simulink model "XY_1_pen_sim"  (R2024b)
settings: Solver=ode4  StartTime=0.0  StopTime=T_run  FixedStep=Ts_plant  RelTol=1e-3
StopFcn:
  | XY_stop
values from neighbouring files (symbols this model uses):
  alpha_s = 0    [XY_setup.m]
  anim_Ts = 0.2    [XY_setup.m]
  animate = 1    [XY_1_pen_sim_run.m]    (also in XY_compare.m = 0; XY_run_all.m; XY_setup.m)
  B_eff = 0.30    (= 0.3)    [XY_setup.m]
  b_trk = 0.28    [XY_setup.m]
  d_reach = 0.03    [XY_setup.m]
  db_v = 47    [XY_setup.m]
  db_w = 20    [XY_setup.m]
  dist_p = [slip_k; wob_amp; wob_f]    [XY_setup.m]
  dyn_p = [m_r; l_trk; b_trk; mu_l; mu_t; N_mag; g_acc]    [XY_setup.m]
  F_max = 200    [XY_setup.m]
  imu_drift = deg2rad(0.02)    [XY_setup.m]
  imu_sigma = deg2rad(0.3)    [XY_setup.m]
  imu_Ts = 0.01    [XY_setup.m]
  K_c = 0    [XY_setup.m]
  K_ci = 0    [XY_setup.m]
  K_dist = 1.0    (= 1)    [XY_setup.m]
  K_ptheta = 1.4    [XY_setup.m]
  k_pwm = v_full/(400 - pwm_dz)    (= 0.000540540540541)    [XY_setup.m]
  K_px = 0.3    [XY_setup.m]
  K_py = 5.0    (= 5)    [XY_setup.m]
  K_yaw = 2.0    (= 2)    [XY_setup.m]
  Ki_v = 15000    [XY_setup.m]
  Ki_w = 15000    [XY_setup.m]
  Kp_v = 1500    [XY_setup.m]
  Kp_w = 1500    [XY_setup.m]
  L_r = sqrt((l_trk^2 + b_trk^2)/12)    [XY_setup.m]
  line_post = 0.04    [XY_setup.m]
  line_pre = 0.06    [XY_setup.m]
  pen_A = [-0.70; 0.30]    [XY_setup.m]
  pen_B = [ 0.50; 0.30]    [XY_setup.m]
  pen_d = r_pen0 - r_tag    [XY_setup.m]
  psi0 = pi/2    (= 1.57079632679)    [XY_setup.m]
  pwm_dz = 30    [XY_setup.m]
  q0 = [-0.85; 0.10; pi/2]    [XY_setup.m]
  q0c = [q0(1:2) - [cos(q0(3)) -sin(q0(3)); sin(q0(3)) cos(q0(3))] * r_tag; q0(3)]    [XY_setup.m]
  r_tag = [-0.080;  0.060]    [XY_setup.m]
  stage_acc = 500    [XY_setup.m]
  stage_c = stage_travel/2    (= 50.8)    [XY_setup.m]
  stage_cmd_Ts = 0.04    [XY_setup.m]
  stage_delay = 0.01    [XY_setup.m]
  stage_Fv_F = [32 32 29 26.5 25 22  20 17.5 14  9]    [XY_setup.m]
  stage_Fv_v = [0  2  7  13  20  32  45  60  80  104]    [XY_setup.m]
  stage_travel = 101.6    [XY_setup.m]
  stage_Ts = 0.05    [XY_setup.m]
  stage_vcmd = 0.8*stage_vmax    (= 83.2)    [XY_setup.m]
  stage_vmax = 104    [XY_setup.m]
  stg_p = [m_sx; m_sy; c_s; Kp_s; Kd_s; Ki_s; g_acc]    [XY_compare.m]    (also in XY_setup.m)
  tau_pred = 0    [XY_setup.m]
  th_tol = deg2rad(1)    [XY_setup.m]
  trk_A = -eye(2)/tau_trk    [XY_setup.m]
  trk_B = eye(2)/tau_trk    [XY_setup.m]
  trk_C = eye(2)    [XY_setup.m]
  trk_D = zeros(2)    [XY_setup.m]
  Ts_ctrl = 0.01    [XY_setup.m]
  v_full = 0.20    (= 0.2)    [XY_setup.m]
  v_max = 0.20    (= 0.2)    [XY_setup.m]
  v_ref = 0.03    [XY_setup.m]
  w_full = 2*k_pwm*(400 - db_w)/B_eff    (= 1.36936936937)    [XY_setup.m]
  w_max = deg2rad(45)    [XY_setup.m]
  x = c(1) + s(1)/2*[-1 1 1 -1 -1 1 1 -1]    [XY_animate.m]
  x_s0 = [stage_c; stage_c; 0; 0; 0; 0] .* [1e-3; 1e-3; 1; 1; 1; 1]    [XY_setup.m]
  x_t0 = [stage_c; stage_c; 0; 0]    [XY_setup.m]
  y = c(2) + s(2)/2*[-1 -1 1 1 -1 -1 1 1]    [XY_animate.m]    (also in build_xy_models.m = q(2))
  zk_delay = 0.05    [XY_setup.m]
  zk_sigma = 0.0010    (= 0.001)    [XY_setup.m]
  zk_Ts = 0.05    [XY_setup.m]
  zk_xsign = -1    [XY_setup.m]
  zk_ywall = 0.02    [XY_setup.m]
undefined symbols (not defined in the file or in its folder): orientation, point, quaternion, twist
libraries: ros2lib x20, simulink x4, slpidlib x2
(part 2 of 2)

== matlab function XY_1_pen_sim/PenCtrl/PenComp ==
  data: lineAB input; s_cmd output; mode input; pose input; pen_d input; stage_c input; pen_on output; sigma output
function [s_cmd, pen_on, sigma] = PenComp(lineAB, mode, pose, pen_d, stage_c)
% PenComp : 펜 기구학 보상. 펜이 직선 위에 오도록 스테이지 위치 명령을 계산한다
% PenComp : pen kinematic compensation. Computes the stage position command that puts the pen on the line
% 입력 / Inputs
%   lineAB  [4x1, m]   [A; B] 펜이 그릴 직선, 벽면 좌표 (x 오른쪽, y 위) / pen line in wall coordinates (x right, y up)
%   mode    [-]        미션 모드. 3 (직선 추종) 일 때만 보상 / mission mode; compensates only in mode 3
%   pose    [3x1: m, m, rad]  측정 태그 자세 [x; y; psi] (Nav) / measured tag pose
%   pen_d   [2x1, m]   태그 -> 펜 레버암, 바디 좌표 [x_B; y_B], 스테이지 중앙일 때 (= d)
%                      tag-to-pen lever arm in body axes, with the stage centred (= d)
%   stage_c [mm]       스테이지 중앙 (50.8, 두 축 같음) / stage centre (50.8 on both axes)
% 출력 / Outputs
%   s_cmd  [2x1, mm]   스테이지 목표 [X; Y] (X = x_B 전진 축, Y = y_B 왼쪽 축), 0-101.6
%                      stage target [X; Y] (X along x_B forward, Y along y_B left) -> /stage/target_pos
%   pen_on [0/1]       1 = 펜 다운 (펜 목표가 A 와 B 사이) / 1 = pen down (pen target between A and B)
%   sigma  [m]         직선 위 진행 거리 (A 에서 0, B 에서 L) / distance travelled along the line
% 원리 / Principle
%   펜 = 태그 + R(psi) (pen_d + (s - s_c)/1000) 을 s 에 대해 푼다. /1000 은 mm -> m.
%   Solve  pen = tag + R(psi) (pen_d + (s - s_c)/1000)  for s.  The 1000 converts m to mm.
%   p_des : 스테이지 중앙일 때 펜 위치 c0 를 직선에 내린 수선의 발
%           foot of the perpendicular from c0 (pen with the stage centred) to the line
%   진행 방향은 로봇이 맡고, 스테이지는 직선과의 어긋남(횡오차 + heading 오차)만 지운다
%   The robot provides the motion along the line; the stage removes only the offset from the line.
A = lineAB(1:2);  B = lineAB(3:4);
L = norm(B - A);  u = (B - A) / max(L, 1e-9);
pT = pose(1:2);
R  = [cos(pose(3)) -sin(pose(3)); sin(pose(3)) cos(pose(3))];
pc = pT + R * pen_d;                 % 스테이지 중앙일 때 펜 위치 / pen position with the stage centred
sigma = dot(u, pc - A);              % 직선 위 진행 거리 / distance along the line
pen_on = 0;
s_cmd = [stage_c; stage_c];
if round(mode) == 3
    % 직선 구간에 들어서면 펜을 내리기 전부터 스테이지를 미리 보낸다 (시작 과도 제거)
    % p_des 는 직선 위 수선의 발 (A, B 로 자르지 않는다): 진행 방향은 로봇이 맡고
    % 스테이지는 직선에서 벗어난 만큼만 지운다. A 로 자르면 펜이 A 앞에 있을 때
    % 남은 진행 거리(line_pre = 60 mm)까지 스테이지가 메우려 해서 행정 끝에 닿는다
%   On entering the line segment the stage is sent ahead even before pen down (removes the start transient).
%   p_des is the foot of the perpendicular on the line (not clipped to A, B): the robot provides the motion
%   along the line and the stage removes only the offset. Clipping to A would make the stage try to cover
%   the remaining run-in (line_pre = 60 mm) while the pen is before A, hitting the end of travel
    p_des = A + sigma * u;
    e_b = R' * (p_des - pT) - pen_d;   % 바디 좌표 펜 이동량 [m] / pen displacement in body frame [m]
    s_cmd = stage_c + 1000 * e_b;
    pen_on = double(sigma >= 0 && sigma <= L);
end

== matlab function XY_1_pen_sim/RobotPlant/EscInv ==
  data: motor_pwm input; v_trk_cmd output; pwm_dz input; k_pwm input
function v_trk_cmd = EscInv(motor_pwm, pwm_dz, k_pwm)
% EscInv : 가상 ESC. PWM -> 궤도 속도 명령 (calc_pwm 의 역) / virtual ESC: PWM -> track speed command
% 입력 / Inputs
%   motor_pwm [2x1, count] /motor_pwm [왼쪽; 오른쪽] / [left; right]
%   pwm_dz [count] ESC 데드존 (30) / ESC dead zone;   k_pwm [m/s per count] 기울기 / slope
% 출력 / Output
%   v_trk_cmd [2x1, m/s]  [vL; vR] 궤도 속도 명령 / track speed commands
% 원리: 우측 반전 해제 -> 데드존 -> count 를 속도로 / undo the right-motor inversion, dead zone, scale
pL =  (motor_pwm(1) - 1500);
pR = -(motor_pwm(2) - 1500);
v_trk_cmd = k_pwm * [sign(pL) * max(0, abs(pL) - pwm_dz);
                     sign(pR) * max(0, abs(pR) - pwm_dz)];

== matlab function XY_1_pen_sim/RobotPlant/SpeedErr ==
  data: v_trk input; e_v output; V_act input; B_eff input; L_r input; e_Lw output
function [e_v, e_Lw] = SpeedErr(v_trk, V_act, B_eff, L_r)
% SpeedErr (운동모델) : 궤도 속도 명령 -> 차체 속도 오차. 6WP 와 같이 둘째 성분은 L*omega 단위
% SpeedErr (plant)    : track speed command -> body speed error; 2nd component in L*omega units as in 6WP
% 입력 / Inputs
%   v_trk [2x1, m/s]  지연을 거친 궤도 속도 명령 [vL; vR] / lagged track speed commands
%   V_act [2x1: m/s, rad/s]  실제 차체 속도 [v; omega] / actual body speed
%   B_eff [m]  조향 유효 궤도 간격 / effective track spacing;   L_r [m]  관성 반경 / radius of gyration
% 출력 / Outputs
%   e_v [m/s] = (vL+vR)/2 - v,   e_Lw [m/s] = L_r ((vR-vL)/B_eff - omega)
v_c = 0.5 * (v_trk(1) + v_trk(2));
w_c = (v_trk(2) - v_trk(1)) / B_eff;
e_v  = v_c - V_act(1);
e_Lw = L_r * (w_c - V_act(2));

== matlab function XY_1_pen_sim/RobotPlant/Control_allocation ==
  data: tau_X input; Fr output; tau_N input; b_trk input; L_r input; Fl output
function [Fr, Fl] = Control_allocation(tau_X, tau_N, b_trk, L_r)
% Control_allocation : 차체 힘·모멘트 -> 좌우 궤도 구동력 (6WP_sim 과 같은 식)
% Control_allocation : body force and moment -> right/left track forces (as in 6WP_sim)
% 입력 / Inputs : tau_X [N] 전진 힘 / surge force;  tau_N [N] 요 모멘트/L / yaw moment divided by L
%                 b_trk [m] 궤도 간격 / track spacing;  L_r [m]
% 출력 / Outputs: Fr, Fl [N] 오른쪽·왼쪽 궤도 구동력 / right and left track forces
% 원리: [tau_X; tau_N] = [1 1; b/2L -b/2L] [Fr; Fl] 를 푼다 / solve this 2x2 system
B_tilde = [1, 1; b_trk/(2*L_r), -b_trk/(2*L_r)];
F = B_tilde \ [tau_X; tau_N];
Fr = F(1);  Fl = F(2);

== matlab function XY_1_pen_sim/RobotPlant/compute_u ==
  data: V_act input; u output; alpha_s input
function u = compute_u(V_act, alpha_s)
% compute_u (6WP_sim) : 회전 중심(ICR)의 길이방향 이동량 / longitudinal shift of the ICR
% 입력 / Inputs : V_act [m/s, rad/s];  alpha_s [rad] ICR 이동각 (0 이면 u = 0) / ICR shift angle
% 출력 / Output : u [m]
R_turn = abs(V_act(1) / max(0.01, abs(V_act(2))));
u = -sign(V_act(2)) * R_turn * sin(alpha_s);

== matlab function XY_1_pen_sim/RobotPlant/Dynamics ==
  data: q input; V_act input; u input; V_dot output; u_dot input; Fr input; Fl input; dyn_p input
function V_dot = Dynamics(q, V_act, u, u_dot, Fr, Fl, dyn_p)
% Dynamics : 궤도차량 동역학 (Zou 2018), 벽면판 / tracked-vehicle dynamics (Zou 2018), wall version
% 입력 / Inputs
%   q [3x1: m, m, rad]  로봇 중심 자세 / robot centre pose;  V_act [2x1: m/s, rad/s] [v; omega]
%   u [m], u_dot [m/s]  ICR 이동량과 그 미분 / ICR shift and its rate
%   Fr, Fl [N]  궤도 구동력 / track forces
%   dyn_p = [m kg; l m; b m; mu_l -; mu_t -; N_mag N; g m/s^2]
% 출력 / Output : V_dot [2x1: m/s^2, rad/s^2]
% 원리 / Principle : M~ nu_dot + C~ nu + S^T (f1 + f2) = B~ tau + S^T f_g,  nu = [v; L omega]
% 6WP_sim Dynamics 와 같은 식 (궤도차량 동역학, 논문 Table 1 모델). 벽면판에서 바꾼 점:
%  (1) 바닥 하중 W -> 자석 흡착력 N_mag : 벽에서 마찰을 만드는 수직력
%  (2) 중력 f_g = [0; -m g; 0] 추가    : 벽면 y = 위
%  (3) 회전 저항 Mr 는 회전을 막는 쪽으로 (l^2/4 - u^2). 6WP 식 (u^2 - l^2/4) 은
%      u = 0 근처에서 회전을 돕는 부호가 되어 헤딩 떨림(stick-slip)을 만든다
%  (4) sign() -> tanh(./eps) : 정지 근처 수치 떨림 방지
% Same equations as 6WP_sim Dynamics (tracked-vehicle dynamics, Table 1 model of the paper). Wall-version changes:
%  (1) ground load W -> magnetic adhesion N_mag : the normal force that creates friction on the wall
%  (2) gravity f_g = [0; -m g; 0] added  : wall y = up
%  (3) turning resistance Mr opposes rotation, (l^2/4 - u^2). The 6WP form (u^2 - l^2/4) assists
%      rotation near u = 0 and causes heading stick-slip
%  (4) sign() -> tanh(./eps) : avoids numerical chatter near standstill
m = dyn_p(1); l = dyn_p(2); b = dyn_p(3); mu_l = dyn_p(4); mu_t = dyn_p(5); N = dyn_p(6); g = dyn_p(7);
L = sqrt((l^2 + b^2)/12);
B_tilde = [1, 1; b/(2*L), -b/(2*L)];
B_tau = B_tilde * [Fr; Fl];
theta = q(3);  v = V_act(1);  omega = V_act(2);
M_mat = m * eye(3);
Rl = mu_l * N / 2;
f1_vec = [2*Rl*cos(theta); 2*Rl*sin(theta); 0] * tanh(v/0.005);
Fy = 2 * tanh(omega/0.01) * mu_t * u * (N / l);
Mr = tanh(omega/0.01) * mu_t * (N / l) * (l^2/4 - u^2);
f2_vec = [Fy*sin(theta); -Fy*cos(theta); Mr/L];
f_g = [0; -m*g; 0];
S_mat = [cos(theta), (u/L)*sin(theta); sin(theta), -(u/L)*cos(theta); 0, 1];
S_dot = [-omega*sin(theta), (u_dot/L)*sin(theta) + (u*omega/L)*cos(theta);
          omega*cos(theta), -(u_dot/L)*cos(theta) + (u*omega/L)*sin(theta); 0, 0];
M_tilde = S_mat' * M_mat * S_mat;
C_tilde = S_mat' * M_mat * S_dot;
V_dot = M_tilde \ (B_tau - C_tilde*[v; L*omega] - S_mat'*f1_vec - S_mat'*f2_vec + S_mat'*f_g);
V_dot(2) = V_dot(2) / L;          % [v_dot; omega_dot]

== matlab function XY_1_pen_sim/Mission/Guards ==
  data: pose input; dist_start output; pen_A input; pen_B input; pen_d input; line_pre input; line_post input; r_tag input; th_err output; along_rem output
function [dist_start, th_err, along_rem] = Guards(pose, pen_A, pen_B, pen_d, line_pre, line_post, r_tag)
% Guards : Stateflow 전이 조건에 쓸 거리·각 (실기 Chart 의 dist, th_err, dist_to_WP2 와 같은 뜻)
% Guards : distances and angle used by the Stateflow transitions (dist, th_err, dist_to_WP2 of the real Chart)
% 입력 / Inputs
%   pose         [3x1: m, m, rad] 측정 태그 자세 [x; y; psi] / measured tag pose
%   pen_A, pen_B [2x1, m]   펜이 그릴 직선의 시작·끝 (벽면) / start and end of the pen line (wall)
%   pen_d        [2x1, m]   태그 -> 펜 레버암, 바디 좌표, 스테이지 중앙일 때 / tag-to-pen lever arm, body frame, stage centred
%   line_pre, line_post [m] 직선 앞뒤로 로봇이 더 가는 거리 / run-in and run-out lengths of the robot segment
%   r_tag        [2x1, m]   로봇 중심 -> 태그, 바디 좌표 / robot centre to tag, body frame
% 출력 / Outputs
%   dist_start [m]   추정 중심과 출발 중심 cA 의 거리 (모드 1 -> 2) / estimated centre to start centre cA (mode 1 -> 2)
%   th_err     [rad] 직선 방향 - heading, [-pi, pi] (모드 2 -> 3) / line direction minus heading (mode 2 -> 3)
%   along_rem  [m]   태그에서 로봇 끝점 rB 까지 남은 진행 거리 (모드 3 -> 4) / distance left to rB along the line (mode 3 -> 4)
th = atan2(pen_B(2) - pen_A(2), pen_B(1) - pen_A(1));   % 펜 직선 방향 / pen line direction
u  = [cos(th); sin(th)];
R  = [cos(th) -sin(th); sin(th) cos(th)];
% 로봇(태그)이 따라갈 선 = 펜 직선을 R*pen_d 만큼 옮긴 것 (스테이지 중앙일 때 펜이 직선 위)
% Line the robot (tag) follows = pen line shifted by R*pen_d (pen on the line when the stage is centred)
rA = pen_A - R*pen_d - u*line_pre;    % 로봇 출발점 (펜이 A 에 닿기 line_pre 전) / robot start (line_pre before the pen reaches A)
rB = pen_B - R*pen_d + u*line_post;   % 로봇 끝점 / robot end point
% 제자리 회전은 중심 둘레로 돈다: 회전 뒤 태그가 rA 에 오려면 중심이 cA 에 있어야 한다
% In-place turns pivot about the centre: for the tag to end at rA the centre must be at cA
cA = rA - R*r_tag;
p = pose(1:2);
Rp = [cos(pose(3)) -sin(pose(3)); sin(pose(3)) cos(pose(3))];
dist_start = norm(cA - (p - Rp*r_tag));                        % 중심과 출발 중심 cA 의 거리 / centre to start centre cA
th_err     = atan2(sin(th - pose(3)), cos(th - pose(3)));      % 직선 방향 오차 / line direction error
along_rem  = dot(rB - p, u);                                   % 끝점까지 남은 진행 거리 / distance left to the end point

== matlab function XY_1_pen_sim/RobotPlant/Kinematics ==
  data: V_act input; q input; u input; q_dot output; t input; dist_p input
function q_dot = Kinematics(V_act, q, u, t, dist_p)
% Kinematics : 차체 속도 -> 중심 자세 변화율 (+ 벽면 외란) / body speed -> centre pose rate (+ wall disturbance)
% 입력 / Inputs : V_act [m/s, rad/s];  q [m, m, rad] 중심 자세 / centre pose;  u [m];  t [s]
%                 dist_p = [slip_k -; 요철 진폭 A rad / wobble amplitude; 주파수 f Hz / frequency]
% 출력 / Output : q_dot [3x1: m/s, m/s, rad/s]
% 6WP_sim Kinematics: q_dot = S_mat * [v; L*omega]  (여기서는 q(3) = psi 로 정리)
% 벽면 외란 (실기 영상·ZeroKey 로그에서 본 현상, [실측 필요]):
%   자석 궤도 크리프 : 이동 속도의 slip_k 배만큼 중력 방향(-y) 으로 밀린다
%   궤도 요철        : heading 이 두 주파수로 조금씩 흔들린다
% 6WP_sim Kinematics: q_dot = S_mat * [v; L*omega]  (written here with q(3) = psi)
% Wall disturbances (seen in real robot videos and ZeroKey logs, [measurement needed]):
%   magnetic track creep : pushed toward gravity (-y) by slip_k times the travel speed
%   track unevenness     : heading wobbles slightly at two frequencies
theta = q(3);  v = V_act(1);  omega = V_act(2);
slip_k = dist_p(1);  A = dist_p(2);  f = dist_p(3);
wob = A*2*pi*f*cos(2*pi*f*t) + 0.5*A*2*pi*(2.3*f)*cos(2*pi*(2.3*f)*t + 1.0);
q_dot = [v*cos(theta) + u*omega*sin(theta);
         v*sin(theta) - u*omega*cos(theta) - slip_k*abs(v);
         omega + wob];

== matlab function XY_1_pen_sim/RobotPlant/TagPoint ==
  data: q_c input; q_tag output; r_tag input
function q_tag = TagPoint(q_c, r_tag)
% TagPoint : 입력 q_c [m, m, rad] 중심 자세, r_tag [2x1, m] -> 출력 q_tag [m, m, rad] 태그 자세 (= q_true)
% TagPoint : input centre pose q_c and r_tag -> output tag pose q_tag (= q_true)
% 중심 -> 태그: p = c + R(psi) r_tag. 회전하면 태그는 반경 |r_tag| 원호를 그린다
% Centre -> tag: p = c + R(psi) r_tag. While turning the tag moves on an arc of radius |r_tag|
R = [cos(q_c(3)) -sin(q_c(3)); sin(q_c(3)) cos(q_c(3))];
q_tag = [q_c(1:2) + R * r_tag; q_c(3)];

== matlab function XY_1_pen_sim/Sensors/ZkWorld ==
  data: q_true input; zk output; zk_ywall input; noise input; zk_xsign input
function zk = ZkWorld(q_true, zk_ywall, noise, zk_xsign)
% ZkWorld : 가상 ZeroKey 위치 / virtual ZeroKey position
% 입력 / Inputs : q_true [m, m, rad] 참 태그 자세 / true tag pose;  zk_ywall [m] 벽 법선 오프셋 / wall-normal offset
%                 noise [3x1, m] 백색 잡음 (sigma 1 mm) / white noise
% 출력 / Output : zk [3x1, m] 월드 [x; y; z] -> 지연 50 ms -> 20 Hz -> /zerokey/position
% 벽면 (x, y) -> ZeroKey 월드 좌표 (x = zk_xsign * 벽면 x, y = 벽 법선 오프셋, z = 벽면 y) + 측정 잡음
% Wall (x, y) -> ZeroKey world (x = zk_xsign * wall x, y = wall-normal offset, z = wall y) + noise
zk = [zk_xsign * q_true(1); zk_ywall; q_true(2)] + noise(:);

== matlab function XY_1_pen_sim/Sensors/ZkVel ==
  data: q_true input; zkv output; V_true input; r_tag input; zk_xsign input
function zkv = ZkVel(q_true, V_true, r_tag, zk_xsign)
% ZkVel : 입력 q_true [m, m, rad], V_true [m/s, rad/s], r_tag [m] -> 출력 zkv [3x1, m/s] -> /zerokey/vel
% ZkVel : inputs q_true, V_true, r_tag -> output zkv [3x1, m/s] world velocity -> /zerokey/vel
% ZeroKey 속도 (월드): x = zk_xsign * 벽면 x, z = 벽면 y. 태그 속도 = 중심 속도 + omega J R r_tag
% ZeroKey velocity (world): x = zk_xsign * wall x, z = wall y. Tag velocity = centre velocity + omega J R r_tag
psi = q_true(3);  R = [cos(psi) -sin(psi); sin(psi) cos(psi)];
pd = V_true(1) * [cos(psi); sin(psi)] + V_true(2) * [0 -1; 1 0] * R * r_tag;
zkv = [zk_xsign * pd(1); 0; pd(2)];

== matlab function XY_1_pen_sim/Sensors/ImuQuat ==
  data: q_true input; quat output; t input; imu_drift input; noise input
function quat = ImuQuat(q_true, t, imu_drift, noise)
% ImuQuat : 입력 q_true [m, m, rad], t [s], imu_drift [rad/s], noise [rad] -> 출력 quat [4x1] (w,x,y,z) -> /imu/data
% ImuQuat : inputs true pose, time, drift rate, noise -> output attitude quaternion -> /imu/data
% IMU 요각 = 참 heading + 드리프트 + 잡음 -> 쿼터니언 (6WP_sim Euler2Quat 와 같은 식)
% IMU yaw = true heading + drift + noise -> quaternion (same as 6WP_sim Euler2Quat)
psi = q_true(3) + imu_drift * t + noise;
quat = [cos(psi/2); 0; 0; sin(psi/2)];

== matlab function XY_1_pen_sim/Sensors/ZkQuat ==
  data: q_true input; quat output; noise input
function quat = ZkQuat(q_true, noise)
% ZkQuat : 입력 q_true, noise [rad] -> 출력 quat [4x1] -> /zerokey/orientation (이 제어기는 쓰지 않음)
% ZkQuat : output quaternion -> /zerokey/orientation (not used by this controller, kept for the real models)
% ZeroKey INS 요각 = 참 heading + 잡음 (드리프트 없음, 대신 IMU 보다 잡음이 크다) -> 쿼터니언
% ZeroKey INS yaw = true heading + noise (no drift, but noisier than the IMU) -> quaternion
psi = q_true(3) + noise;
quat = [cos(psi/2); 0; 0; sin(psi/2)];

== matlab function XY_1_pen_sim/StagePlant/ZaberTraj ==
  data: s_goal input; x_t_dot output; x_t input; stage_vmax input; stage_acc input; stage_travel input
function x_t_dot = ZaberTraj(s_goal, x_t, stage_vmax, stage_acc, stage_travel)
% ZaberTraj : Zaber 펌웨어 궤적 생성기의 모델 (사용자가 바꿀 수 없는 상용 부분)
% ZaberTraj : model of the Zaber firmware trajectory generator (commercial, not ours to change)
% 입력 / Inputs : s_goal [2x1, mm] move abs 목표 / move abs target;  x_t [4x1: mm, mm, mm/s, mm/s]
%                 stage_vmax [mm/s] maxspeed;  stage_acc [mm/s^2] accel;  stage_travel [mm] 행정 / travel
% 출력 / Output : x_t_dot [4x1: mm/s, mm/s, mm/s^2, mm/s^2]
% Zaber 펌웨어의 move abs 궤적 (두 축 따로).  상태 x_t = [s_t(2) mm; v_t(2) mm/s]
%   목표까지 남은 거리에서 멈출 수 있는 속도 sqrt(2 a |e|) 와 maxspeed 중 작은 값으로 간다
%   (가속·감속 한계 = accel 설정).  새 move abs 가 오면 그 자리에서 목표만 바뀐다
% Zaber firmware move abs trajectory (each axis separately).  State x_t = [s_t(2) mm; v_t(2) mm/s]
%   Moves at the smaller of maxspeed and the speed sqrt(2 a |e|) that can still stop at the target
%   (acceleration/deceleration limit = accel setting).  A new move abs only changes the target in place
goal = min(max(s_goal(:), 0), stage_travel);
s = x_t(1:2);  v = x_t(3:4);
e = goal - s;
v_des = sign(e) .* min(stage_vmax, sqrt(2*stage_acc*abs(e)));
a = min(max(50*(v_des - v), -stage_acc), stage_acc);
x_t_dot = [v; a];

== matlab function XY_1_pen_sim/StagePlant/ZaberServo ==
  data: x_t input; x_dot output; x_s input; q_true input; stg_p input; Fv_v input; Fv_F input
function x_dot = ZaberServo(x_t, x_s, q_true, stg_p, Fv_v, Fv_F)
% ZaberServo : Zaber 내부 위치 서보 + 캐리지 질량의 모델 (상용 펌웨어, 명령만 줄 수 있음)
% ZaberServo : model of the internal Zaber position servo and carriage mass (commercial; command only)
% 입력 / Inputs : x_t [mm, mm/s] 궤적 / trajectory;  x_s [6x1: m, m, m/s, m/s, m s, m s] 캐리지 상태 / carriage state
%                 q_true [m, m, rad] (중력 방향 계산 / for the gravity direction)
%                 stg_p = [m_X kg; m_Y kg; c N s/m; Kp N/m (2); Kd N s/m (2); Ki N/(m s) (2); g m/s^2]
%                 Fv_v [mm/s], Fv_F [N]  추력-속도 곡선 / thrust-speed curve
% 출력 / Output : x_dot [6x1: m/s, m/s, m/s^2, m/s^2, m, m]
% Zaber X-LSM100B 두 축 (X = 아래 축, Y = 위 축).  상태 x_s = [s(2) m; v(2) m/s; 적분(2)]
%   스테퍼는 궤적을 단단한 스프링처럼 따라간다 -> 높은 대역의 위치 루프로 나타낸다
%   낼 수 있는 힘은 속도에 따라 줄어든다 (데이터시트 Thrust-Speed, B 형 24 V 곡선 Fv_v -> Fv_F)
%   X 축은 Y 축 스테이지 전체 + 펜 홀더를 민다 (m_sx > m_sy)
%   벽면 중력 [0; -g] 를 바디 좌표로 돌려 각 축에 m g 성분을 건다
% Two-axis Zaber X-LSM100B (X = lower axis, Y = upper axis).  State x_s = [s(2) m; v(2) m/s; integral(2)]
%   The stepper follows the trajectory like a stiff spring -> modelled as a high-bandwidth position loop
%   Available force drops with speed (datasheet Thrust-Speed, type B 24 V curve Fv_v -> Fv_F)
%   The X axis pushes the whole Y-axis stage + pen holder (m_sx > m_sy)
%   Wall gravity [0; -g] is rotated into the body frame and its m g component applied on each axis
m  = stg_p(1:2);  c = stg_p(3);
Kp = stg_p(4:5);  Kd = stg_p(6:7);  Ki = stg_p(8:9);  g = stg_p(10);
s = x_s(1:2);  v = x_s(3:4);  ie = x_s(5:6);
s_t = x_t(1:2)/1000;  v_t = x_t(3:4)/1000;
e = s_t - s;
F_av = interp1(Fv_v, Fv_F, min(abs(v)*1000, Fv_v(end)));   % 지금 속도에서 낼 수 있는 추력 [N] / thrust available at the current speed [N]
F = min(max(Kp.*e + Ki.*ie + Kd.*(v_t - v), -F_av), F_av);
psi = q_true(3);
g_b = [cos(psi) sin(psi); -sin(psi) cos(psi)] * [0; -g];
a = (F + m.*g_b - c*v) ./ m;
x_dot = [v; a; e];

== matlab function XY_1_pen_sim/StagePlant/Encoder ==
  data: x_s input; stage_pos output; stage_travel input
function stage_pos = Encoder(x_s, stage_travel)
% Encoder : 입력 x_s [m, m/s, m s], stage_travel [mm] -> 출력 stage_pos [2x1, mm] -> /stage/pos (20 Hz)
% Encoder : output = position reported by get pos [mm], clipped at the travel ends
% 내장 엔코더 위치 [mm] (get pos 가 돌려주는 값), 행정 끝에서 막힌다
stage_pos = min(max(1000 * x_s(1:2), 0), stage_travel);

== matlab function XY_1_pen_sim/PenTrace/PenTraceFcn ==
  data: q_true input; pen_true output; stage_pos input; lineAB input; pen_d input; stage_c input; pen_nocomp output; e_pen output; e_nocomp output
function [pen_true, pen_nocomp, e_pen, e_nocomp] = PenTraceFcn(q_true, stage_pos, lineAB, pen_d, stage_c)
% PenTraceFcn : 참값으로 계산한 펜 위치와 횡오차 (평가 전용, 제어기는 모름)
% PenTraceFcn : true pen position and cross error from true values (evaluation only)
% 입력 / Inputs : q_true [m, m, rad] 참 태그 자세 / true tag pose;  stage_pos [2x1, mm] 엔코더 / encoder;  lineAB [4x1, m];
%                 pen_d [2x1, m];  stage_c [mm]
% 출력 / Outputs: pen_true, pen_nocomp [2x1, m];  e_pen, e_nocomp [m]
% pen_true   : 스테이지가 실제로 움직인 결과의 펜 위치 [x; y] (벽면)
%              pen position [x; y] resulting from the actual stage motion (wall frame)
% pen_nocomp : 스테이지를 중앙에 고정했을 때 펜 위치 (보상 없음 비교)
%              pen position with the stage held at centre (no-compensation comparison)
% e_*        : 직선에 대한 부호 있는 횡오차 [m] (직선 진행방향의 왼쪽 +)
%              signed cross error to the line [m] (left of the line direction +)
A = lineAB(1:2);  B = lineAB(3:4);
u = (B - A) / max(norm(B - A), 1e-9);  n = [-u(2); u(1)];
pT = q_true(1:2);
R  = [cos(q_true(3)) -sin(q_true(3)); sin(q_true(3)) cos(q_true(3))];
pen_true   = pT + R * (pen_d + (stage_pos - stage_c) / 1000);
pen_nocomp = pT + R * pen_d;
e_pen    = dot(n, pen_true - A);
e_nocomp = dot(n, pen_nocomp - A);

== matlab function XY_1_pen_sim/Animate/AnimateFcn ==
  data: q_true input; ok output; pen_true input; pen_on input; stage_pos input; lineAB input; e_pen input; v_cmd input; w_cmd input; V_true input; mode input; t input; en input
function ok = AnimateFcn(q_true, pen_true, pen_on, stage_pos, lineAB, e_pen, v_cmd, w_cmd, V_true, mode, t, en)
%#codegen
% Live plot while the model runs. A MATLAB Function block cannot
% plot, so the drawing function is declared extrinsic: Simulink
% calls plain MATLAB instead of generating code for it.
coder.extrinsic('XY_animate');
ok = 1;
if en > 0.5
    XY_animate(q_true, pen_true, pen_on, stage_pos, lineAB, e_pen, v_cmd, w_cmd, V_true, mode, t);
end

== matlab function XY_1_pen_sim/Nav/NavFcn ==
  settings: updateMethod=DISCRETE  sampleTime=Ts_ctrl
  data: zerokey_position input; pose output; zerokey_vel input; imu_quat input; psi0 input; tau_pred input; zk_xsign input
function pose = NavFcn(zerokey_position, zerokey_vel, imu_quat, psi0, tau_pred, zk_xsign)
% NavFcn : 센서 토픽 -> 측정 자세 (항법)
% NavFcn : sensor topics -> measured pose (navigation)
% 입력 / Inputs
%   zerokey_position [3x1, m]   /zerokey/position point.(x,y,z). 태그 월드 좌표: x 벽 수평, y 벽 법선, z 높이
%                               tag world position: x horizontal, y wall normal, z height
%   zerokey_vel      [3x1, m/s] /zerokey/vel twist.linear.(x,y,z). 태그 월드 속도 / tag world velocity
%   imu_quat         [4x1, -]   /imu/data orientation (w,x,y,z). Xsens 자세 쿼터니언 / Xsens attitude quaternion
%   psi0             [1, rad]   출발 heading (오른쪽 0, 천장 pi/2) / initial heading (0 = right, pi/2 = up)
%   tau_pred         [1, s]     ZeroKey 지연 보상 시간 (0 = 끔) / ZeroKey latency compensation (0 = off)
%   zk_xsign         [-1 / +1]  ZeroKey x 방향: -1 = 벽 정면에서 왼쪽 +, +1 = 오른쪽 + / ZeroKey x: -1 left +, +1 right +
% 출력 / Output
%   pose [3x1: m, m, rad]  [x; y; psi] = 태그 벽면 위치 (x 오른쪽 +, y 위 +) + heading (x 축에서 반시계)
%                          [x; y; psi] = tag position on the wall (x right, y up) + heading (CCW from x)
% 원리 / Principle
%   벽면 x = zk_xsign * ZeroKey x, 벽면 y = ZeroKey z (REP-103 형: z 가 벽 바깥인 오른손 좌표계).
%   철판 벽에서는 자력계를 못 쓰므로 heading 은 첫 유효 샘플의 요각을 0 으로 잡은 상대 요각에 psi0 를 더한 값이다.
%   Wall x = zk_xsign * ZeroKey x, wall y = ZeroKey z (REP-103 style, right-handed with z out of the wall).
%   The steel wall disturbs the magnetometer, so heading is the yaw relative to the first valid sample, plus psi0.
persistent yaw0 ok
if isempty(ok), ok = false; yaw0 = 0; end
qw = imu_quat(1); qx = imu_quat(2); qy = imu_quat(3); qz = imu_quat(4);
yaw = atan2(2*(qw*qz + qx*qy), 1 - 2*(qy*qy + qz*qz));
if ~ok && (abs(qw) + abs(qx) + abs(qy) + abs(qz)) > 0.5
    yaw0 = yaw;  ok = true;
end
a = yaw - yaw0 + psi0;
pose = [zk_xsign * zerokey_position(1); zerokey_position(3); atan2(sin(a), cos(a))];
% ZeroKey 지연 보상 (tau_pred = 0 이면 끔): 측정 속도로 tau_pred 만큼 앞으로 내다본다
% ZeroKey latency compensation (off when tau_pred = 0): predicts ahead by tau_pred with the measured velocity
pose(1:2) = pose(1:2) + tau_pred * [zk_xsign * zerokey_vel(1); zerokey_vel(3)];

== stateflow chart XY_1_pen_sim/Mission/ModeChart ==
  settings: updateMethod=DISCRETE  sampleTime=Ts_ctrl
  state Goto_Start
    entry:
    mode = 1;
  state Turning
    entry:
    mode = 2;
  state Line_Tracking
    entry:
    mode = 3;
    t_line = t;
  state Stop_Destination
    entry:
    mode = 4;
  state Done
    entry:
    done = 1;
  (default) -> Goto_Start
  Goto_Start -> Turning : [dist_start < d_reach]
  Turning -> Line_Tracking : after(1.0,sec)[abs(th_err) < th_tol]
  Line_Tracking -> Stop_Destination : [along_rem < d_reach]
  Stop_Destination -> Done : after(2.0,sec)
  data: dist_start input; th_err input; along_rem input; t input; mode output double =1; t_line output double =0; done output double =0; d_reach parameter; th_tol parameter

== matlab function XY_1_pen_sim/Mission/Waypoints ==
  data: mode input; WP_prev output; pen_A input; pen_B input; pen_d input; line_pre input; line_post input; r_tag input; WP_target output; lineAB output
function [WP_prev, WP_target, lineAB] = Waypoints(mode, pen_A, pen_B, pen_d, line_pre, line_post, r_tag)
% Waypoints : 모드에 따라 로봇이 따라갈 선분을 낸다 (6WP waypoint_manager 역할)
% Waypoints : gives the segment the robot follows in each mode (role of the 6WP waypoint_manager)
% 입력 / Inputs
%   mode [-]  1 출발점 이동, 2 회전, 3 직선 추종, 4 정지, 5 종료 / 1 go to start, 2 turn, 3 line, 4 stop, 5 done
%   pen_A, pen_B, pen_d, line_pre, line_post, r_tag : Guards 와 같음 / same as Guards
% 출력 / Outputs
%   WP_prev   [2x1, m] 태그 선분 시작 rA (펜이 A 에 닿기 line_pre 전) / tag segment start rA
%   WP_target [2x1, m] 모드 1: 출발 중심 cA (중심 기준), 그 뒤: 태그 선분 끝 rB
%                      mode 1: start centre cA (centre-referenced); afterwards: tag segment end rB
%   lineAB    [4x1, m] [A; B] 펜 직선 (PenComp 로 간다) / pen line, sent to PenComp
% 원리 / Principle
%   스테이지가 중앙일 때 펜이 직선 위에 오도록, 태그가 갈 선분은 펜 직선을 R(theta_l) pen_d 만큼 옮긴 것이다.
%   The tag segment is the pen line shifted by -R(theta_l) pen_d, so that the pen is on the line when the stage is centred.
th = atan2(pen_B(2) - pen_A(2), pen_B(1) - pen_A(1));   % 펜 직선 방향 / pen line direction
u  = [cos(th); sin(th)];
R  = [cos(th) -sin(th); sin(th) cos(th)];
% 로봇(태그)이 따라갈 선 = 펜 직선을 R*pen_d 만큼 옮긴 것 (스테이지 중앙일 때 펜이 직선 위)
% Line the robot (tag) follows = pen line shifted by R*pen_d (pen on the line when the stage is centred)
rA = pen_A - R*pen_d - u*line_pre;    % 로봇 출발점 (펜이 A 에 닿기 line_pre 전) / robot start (line_pre before the pen reaches A)
rB = pen_B - R*pen_d + u*line_post;   % 로봇 끝점 / robot end point
% 제자리 회전은 중심 둘레로 돈다: 회전 뒤 태그가 rA 에 오려면 중심이 cA 에 있어야 한다
% In-place turns pivot about the centre: for the tag to end at rA the centre must be at cA
cA = rA - R*r_tag;
WP_prev = rA;
if round(mode) <= 1
    WP_target = cA;
else
    WP_target = rB;
end
lineAB = [pen_A; pen_B];

== matlab function XY_1_pen_sim/RobotCtrl/M1_GotoStart/Fcn1_GotoStart ==
  data: WP_target input; v output; pose input; K_dist input; K_yaw input; r_tag input; w output
function [v, w] = Goto_Start_Position(WP_target, pose, K_dist, K_yaw, r_tag)
% 모드 1 : 6WP_sim Goto_Start_Position, Method 2 (리아프노프형). 6WP 와 같이 로봇 중심을 목표로 보낸다
% Mode 1 : 6WP_sim Goto_Start_Position, Method 2. Drives the robot centre (as in 6WP_sim) to the target
% 입력 / Inputs
%   WP_target [2x1, m]   출발 중심 cA (벽면) / start centre cA (wall)
%   pose      [3x1: m, m, rad] 측정 태그 자세 / measured tag pose
%   K_dist    [1/s]  거리 게인 / distance gain;   K_yaw [1/s]  방향 게인 / bearing gain
%   r_tag     [2x1, m]  중심 -> 태그 (바디) / centre to tag (body)
% 출력 / Outputs
%   v [m/s]   전진 속도 명령 / forward speed command;   w [rad/s] 요 각속도 명령 (반시계 +) / yaw-rate command (CCW +)
% 원리 / Principle
%   v = K_dist rho max(0, cos a), w = K_yaw a + 0.5 sin a cos a. a = 목표 방위 - heading.
%   방향이 90 도 넘게 틀리면 서서 돌기만 한다 / turns on the spot while the bearing error exceeds 90 deg
c = pose(1:2) - [cos(pose(3)) -sin(pose(3)); sin(pose(3)) cos(pose(3))] * r_tag;   % 중심 추정 / centre estimate
err_x = WP_target(1) - c(1);  err_y = WP_target(2) - c(2);
dist = hypot(err_x, err_y);
target_th = atan2(err_y, err_x);
a = atan2(sin(target_th - pose(3)), cos(target_th - pose(3)));
v = K_dist * dist * max(0, cos(a));            % 방향이 맞을 때만 전진 / forward only when roughly aligned
w = K_yaw * a + 0.5 * sin(a) * cos(a);         % 비선형 감쇠항 / nonlinear damping term

== matlab function XY_1_pen_sim/RobotCtrl/M2_Turn/Fcn2_Turn ==
  data: WP_prev input; v output; WP_target input; pose input; K_yaw input; w output
function [v, w] = Turning_Straight_Mode(WP_prev, WP_target, pose, K_yaw)
% 모드 2 : 6WP_sim Turning_Straight_Mode — 제자리 회전으로 heading 을 직선 방향에 맞춘다
% Mode 2 : 6WP_sim Turning_Straight_Mode — turns on the spot until the heading matches the line
% 입력 / Inputs
%   WP_prev, WP_target [2x1, m] 태그 선분 rA, rB / tag segment;  pose [m, m, rad];  K_yaw [1/s]
% 출력 / Outputs
%   v = 0 [m/s],  w = K_yaw wrap(theta_l - psi) [rad/s]
th_final = atan2(WP_target(2) - WP_prev(2), WP_target(1) - WP_prev(1));
th_err = atan2(sin(th_final - pose(3)), cos(th_final - pose(3)));
v = 0;
w = K_yaw * th_err;
